simulink model "drone_plant"  (R2026a)
settings: Solver=ode4  StopTime=inf  FixedStep=P.Ts  RelTol=1e-8
PreLoadFcn:
  | model_params
values from neighbouring files (symbols this model uses):
  P = evalin('base','P')    [drone_panel.m]    (also in record_mission.m)
  x0 = zeros(12,1);  x0(3) = -3    [drone_panel.m]    (also in model_params.m = zeros(12,1); record_mission.m = zeros(12,1);  x0(3) = -P.field.alt)
undefined symbols (not defined in the file or in its folder): forces_islfcn, mixer_islfcn, obs_islfcn, plant_islfcn, pos_att_ctrl_islfcn, poserr_islfcn, sensors_islfcn, spray_islfcn, tilt_islfcn, traj_islfcn, wind_islfcn
settings Model: Creator=MALEK  LastModifiedBy=MALEK
settings SFSimCC: SimGPUStackLimitPerThread=51200
settings RTWCC: GPUStackLimitPerThread=51200

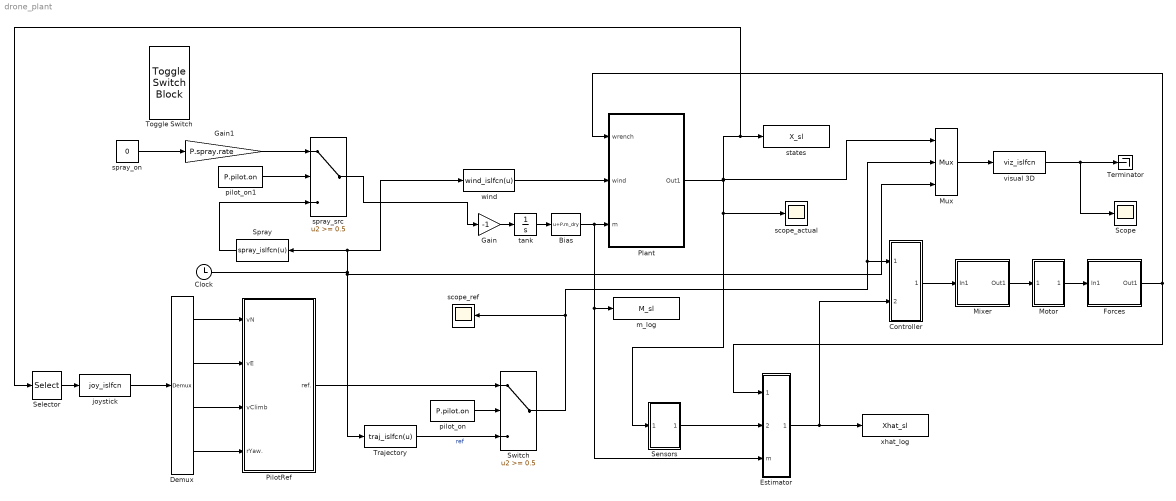
== system drone_plant ==
  Bias : Bias  Bias=P.m_dry  SaturateOnIntegerOverflow=off
  Clock : Clock
  Controller : Subsystem
  Demux : Demux
  Estimator : Subsystem
  Forces : Subsystem
  Gain : Gain  Gain=-1
  Gain1 : Gain  Gain=P.spray.rate
  Mixer : Subsystem
  "Motor  " : Subsystem
  Mux : Mux  Inputs=3
  PilotRef : Subsystem
  Plant : Subsystem
  Scope : Scope
      settings: ActiveDisplayYMinimum=-1  ActiveDisplayYMaximum=1  DataLoggingVariableName=ScopeData2
  Selector : Selector  InputPortWidth=12  IndexOptions=Index vector (dialog)  Indices=9  OutputSizes=1  RuntimeRangeChecks=off
  Sensors : Subsystem
  Spray : MATLABFcn  MATLABFcn=spray_islfcn(u)  OutputDimensions=1
  Switch : Switch  Threshold=0.5  SaturateOnIntegerOverflow=off  InputSameDT=off
  Terminator : Terminator
  Toggle Switch : ToggleSwitchBlock
  Trajectory : MATLABFcn  MATLABFcn=traj_islfcn(u)  OutputDimensions=10
  joystick : MATLABFcn  MATLABFcn=joy_islfcn  OutputDimensions=4
  m_log : ToWorkspace  VariableName=M_sl  SampleTime=-1
  pilot_on : Constant  Value=P.pilot.on
  pilot_on1 : Constant  Value=P.pilot.on
  scope_actual : Scope
      settings: ActiveDisplayYMinimum=-1  ActiveDisplayYMaximum=1
  scope_ref : Scope
      settings: ActiveDisplayYMinimum=-29.000000000000604  ActiveDisplayYMaximum=20.999999999998604
  spray_on : Constant  Value=0
  spray_src : Switch  Threshold=0.5  SaturateOnIntegerOverflow=off  InputSameDT=off
  states : ToWorkspace  VariableName=X_sl  SampleTime=-1
  tank : Integrator  InitialCondition=P.tank_full  LimitOutput=on  UpperSaturationLimit=P.tank_full  LowerSaturationLimit=0
  visual 3D : MATLABFcn  MATLABFcn=viz_islfcn  OutputDimensions=1
  wind : MATLABFcn  MATLABFcn=wind_islfcn(u)  OutputDimensions=3
  xhat_log : ToWorkspace  VariableName=Xhat_sl  SampleTime=-1
  wires:
  Estimator/1(Out1) -> xhat_log/1, Controller/2(In2)
  Sensors/1(Out1) -> Estimator/2(In2)
  Controller/1(Out1) -> Mixer/1(In1)
  Mixer/1(Out1) -> "Motor  "/1(In1)
  Forces/1(Out1) -> Estimator/1(In1), Plant/1(wrench)
  "Motor  "/1(Out1) -> Forces/1(In1)
  Clock/1 -> Trajectory/1, Mux/3, wind/1, Spray/1
  wind/1 -> Plant/2(wind)
  Spray/1 -> spray_src/3
  Gain/1 -> tank/1
  tank/1 -> Bias/1
  Bias/1 -> Estimator/3(m), m_log/1, Plant/3(m)
  PilotRef/1(ref.) -> Switch/1
  pilot_on/1 -> Switch/2
  Trajectory/1 -> Switch/3  "ref"
  Switch/1 -> Controller/1(In1), Mux/2, scope_ref/1
  spray_on/1 -> Gain1/1
  Gain1/1 -> spray_src/1
  spray_src/1 -> Gain/1
  pilot_on1/1 -> spray_src/2
  Mux/1 -> visual 3D/1
  visual 3D/1 -> Scope/1, Terminator/1
  Demux/4 -> PilotRef/4(rYaw.)
  Demux/3 -> PilotRef/3(vClimb)
  Demux/2 -> PilotRef/2(vE)
  Demux/1 -> PilotRef/1(vN)
  joystick/1 -> Demux/1
  Selector/1 -> joystick/1
  Plant/1(Out1) -> Mux/1, Selector/1, states/1, scope_actual/1, Sensors/1(In1)

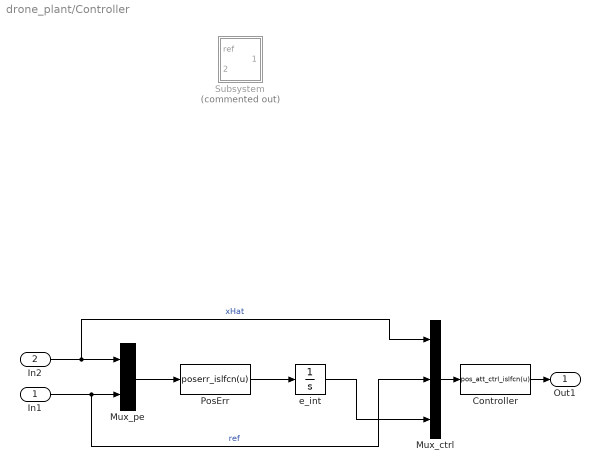
== system drone_plant/Controller ==
  In1 : Inport
  In2 : Inport  Port=2
  Controller : MATLABFcn  MATLABFcn=pos_att_ctrl_islfcn(u)  OutputDimensions=4
  Mux_ctrl : Mux  Inputs=3
  Mux_pe : Mux  Inputs=2
  PosErr : MATLABFcn  MATLABFcn=poserr_islfcn(u)  OutputDimensions=3
  Subsystem : Subsystem  Commented=on
  e_int : Integrator  LimitOutput=on  UpperSaturationLimit=P.int_limit  LowerSaturationLimit=-P.int_limit
  Out1 : Outport
  wires:
  In2/1 -> Mux_ctrl/1, Mux_pe/1  "xHat"
  In1/1 -> Mux_ctrl/2, Mux_pe/2  "ref"
  Mux_pe/1 -> PosErr/1
  PosErr/1 -> e_int/1
  e_int/1 -> Mux_ctrl/3
  Mux_ctrl/1 -> Controller/1
  Controller/1 -> Out1/1

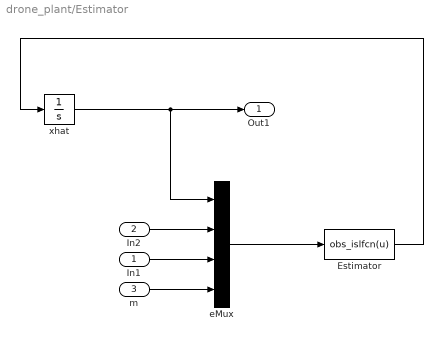
== system drone_plant/Estimator ==
  In1 : Inport
  In2 : Inport  Port=2
  m : Inport  Port=3
  Estimator : MATLABFcn  MATLABFcn=obs_islfcn(u)  OutputDimensions=12
  eMux : Mux
  xhat : Integrator  InitialCondition=x0
  Out1 : Outport
  wires:
  Estimator/1 -> xhat/1
  xhat/1 -> eMux/1, Out1/1
  In2/1 -> eMux/2
  eMux/1 -> Estimator/1
  In1/1 -> eMux/3
  m/1 -> eMux/4

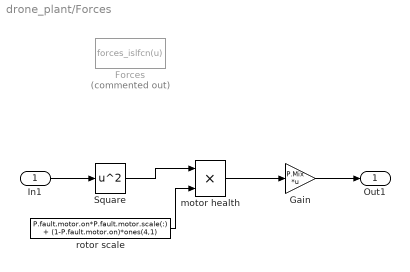
== system drone_plant/Forces ==
  In1 : Inport
  Forces : MATLABFcn  Commented=on  MATLABFcn=forces_islfcn(u)  OutputDimensions=4
  Gain : Gain  Gain=P.Mix  Multiplication=Matrix(K*u)
  Square : Math  Operator=square
  motor health : Product
  rotor scale : Constant  Value=P.fault.motor.on*P.fault.motor.scale(:) + (1-P.fault.motor.on)*ones(4,1)
  Out1 : Outport
  wires:
  In1/1 -> Square/1
  Gain/1 -> Out1/1
  Square/1 -> motor health/1
  rotor scale/1 -> motor health/2
  motor health/1 -> Gain/1

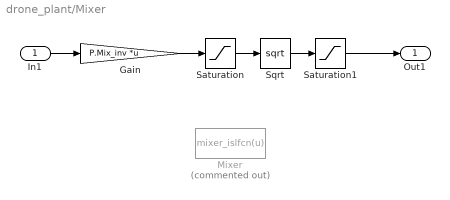
== system drone_plant/Mixer ==
  In1 : Inport
  Gain : Gain  Gain=P.Mix_inv  Multiplication=Matrix(K*u)
  Mixer : MATLABFcn  Commented=on  MATLABFcn=mixer_islfcn(u)  OutputDimensions=4
  Saturation : Saturate  UpperLimit=inf  LowerLimit=0
  Saturation1 : Saturate  UpperLimit=P.omega_max  LowerLimit=P.omega_min
  Sqrt : Sqrt
  Out1 : Outport
  wires:
  In1/1 -> Gain/1
  Gain/1 -> Saturation/1
  Saturation/1 -> Sqrt/1
  Sqrt/1 -> Saturation1/1
  Saturation1/1 -> Out1/1

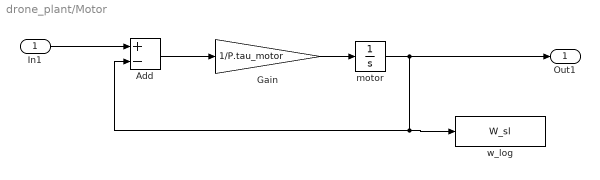
== system drone_plant/Motor   ==
  In1 : Inport
  Add : Sum  Inputs=+-
  Gain : Gain  Gain=1/P.tau_motor
  motor : Integrator  InitialCondition=P.omega_hover*ones(4,1)
  w_log : ToWorkspace  VariableName=W_sl  SampleTime=-1
  Out1 : Outport
  wires:
  In1/1 -> Add/1
  Gain/1 -> motor/1
  motor/1 -> w_log/1, Add/2, Out1/1
  Add/1 -> Gain/1

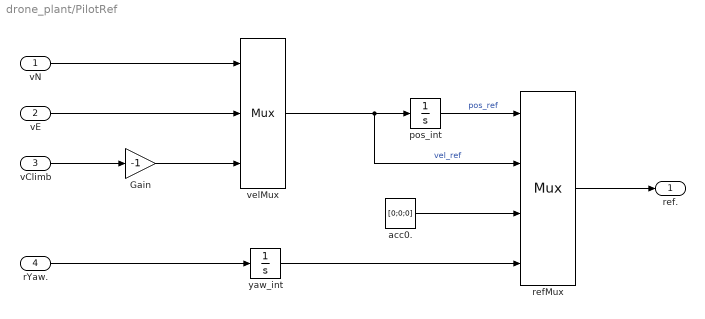
== system drone_plant/PilotRef ==
  vN : Inport
  vE : Inport  Port=2
  vClimb : Inport  Port=3
  rYaw. : Inport  Port=4
  Gain : Gain  Gain=-1
  acc0. : Constant  Value=[0;0;0]
  pos_int : Integrator  InitialCondition=x0(1:3)
  refMux : Mux
  velMux : Mux  Inputs=3
  yaw_int : Integrator  InitialCondition=x0(9)
  ref. : Outport
  wires:
  vClimb/1 -> Gain/1
  Gain/1 -> velMux/3
  vE/1 -> velMux/2
  vN/1 -> velMux/1
  velMux/1 -> refMux/2, pos_int/1  "vel_ref"
  rYaw./1 -> yaw_int/1
  pos_int/1 -> refMux/1  "pos_ref"
  acc0./1 -> refMux/3
  yaw_int/1 -> refMux/4
  refMux/1 -> ref./1

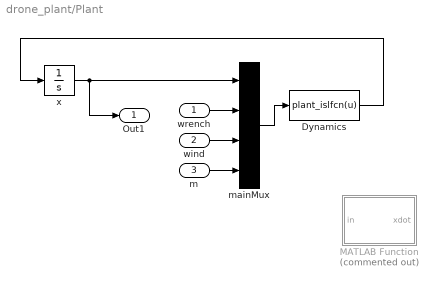
== system drone_plant/Plant ==
  wrench : Inport
  wind : Inport  Port=2
  m : Inport  Port=3
  Dynamics : MATLABFcn  MATLABFcn=plant_islfcn(u)  OutputDimensions=12
  MATLAB Function : MATLAB Function  Commented=on  TreatAsAtomicUnit=on
  mainMux : Mux
  x : Integrator  InitialCondition=x0
  Out1 : Outport
  wires:
  wrench/1 -> mainMux/2
  x/1 -> mainMux/1, Out1/1
  Dynamics/1 -> x/1
  mainMux/1 -> Dynamics/1
  wind/1 -> mainMux/3
  m/1 -> mainMux/4

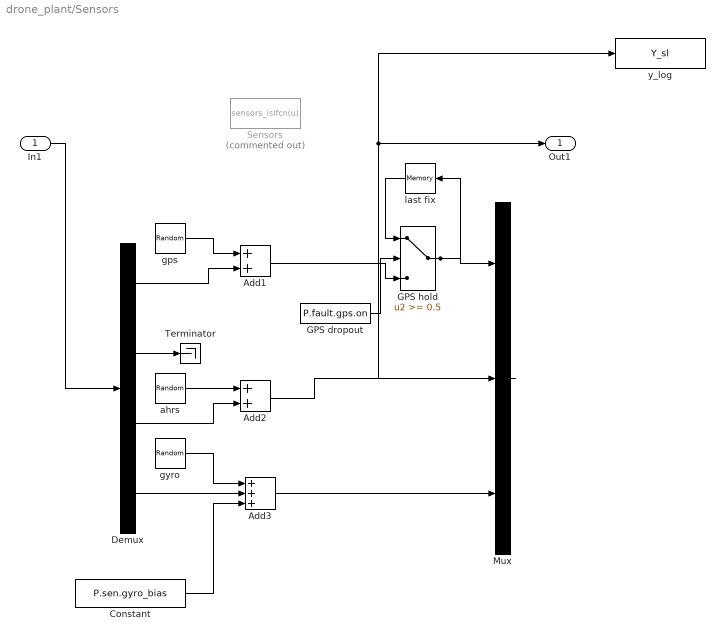
== system drone_plant/Sensors ==
  In1 : Inport
  Add1 : Sum
  Add2 : Sum
  Add3 : Sum  Inputs=+++
  Constant : Constant  Value=P.sen.gyro_bias
  Demux : Demux  Outputs=[3 3 3 3]
  GPS dropout : Constant  Value=P.fault.gps.on
  GPS hold : Switch  Threshold=0.5  SaturateOnIntegerOverflow=off  InputSameDT=off
  Mux : Mux  Inputs=3
  Sensors : MATLABFcn  Commented=on  MATLABFcn=sensors_islfcn(u)  OutputDimensions=9
  Terminator : Terminator
  ahrs : RandomNumber  Mean=[0;0;0]  Variance=P.sen.att_std^2  Seed=23456  SampleTime=P.Ts
  "gps " : RandomNumber  Mean=[0;0;0]  Variance=P.sen.gps_std^2  Seed=12345  SampleTime=P.Ts
  gyro : RandomNumber  Mean=[0;0;0]  Variance=P.sen.gyro_std^2  Seed=34567  SampleTime=P.Ts
  last fix : Memory
  y_log : ToWorkspace  VariableName=Y_sl  SampleTime=-1
  Out1 : Outport
  wires:
  In1/1 -> Demux/1
  Demux/2 -> Terminator/1
  "gps "/1 -> Add1/1
  Demux/1 -> Add1/2
  ahrs/1 -> Add2/1
  Demux/3 -> Add2/2
  gyro/1 -> Add3/1
  Demux/4 -> Add3/2
  Constant/1 -> Add3/3
  Add2/1 -> Mux/2
  Add3/1 -> Mux/3
  Mux/1 -> y_log/1, Out1/1
  Add1/1 -> GPS hold/3
  GPS dropout/1 -> GPS hold/2
  last fix/1 -> GPS hold/1
  GPS hold/1 -> last fix/1, Mux/1

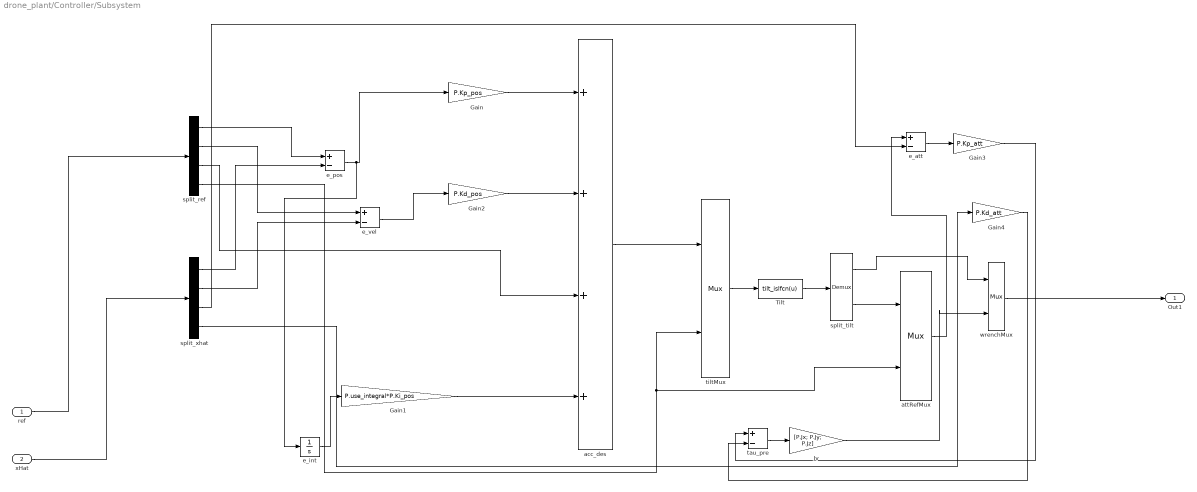
== system drone_plant/Controller/Subsystem ==
  ref : Inport
  xHat : Inport  Port=2
  Gain : Gain  Gain=P.Kp_pos
  Gain1 : Gain  Gain=P.use_integral*P.Ki_pos
  Gain2 : Gain  Gain=P.Kd_pos
  Gain3 : Gain  Gain=P.Kp_att
  Gain4 : Gain  Gain=P.Kd_att
  Jv : Gain  Gain=[P.Jx; P.Jy; P.Jz]
  Tilt : MATLABFcn  MATLABFcn=tilt_islfcn(u)  OutputDimensions=3
  acc_des : Sum  Inputs=++++
  attRefMux : Mux  Inputs=2
  e_att : Sum  Inputs=+-
  e_int : Integrator  LimitOutput=on  UpperSaturationLimit=P.int_limit  LowerSaturationLimit=-P.int_limit
  e_pos : Sum  Inputs=+-
  e_vel : Sum  Inputs=+-
  split_ref : Demux  Outputs=[3 3 3 1]
  split_tilt : Demux  Outputs=[1 2]
  split_xhat : Demux  Outputs=[3 3 3 3]
  tau_pre : Sum  Inputs=+-
  tiltMux : Mux  Inputs=2
  wrenchMux : Mux  Inputs=2
  Out1 : Outport
  wires:
  split_xhat/1 -> e_pos/2
  e_pos/1 -> e_int/1, Gain/1
  attRefMux/1 -> e_att/1
  split_xhat/3 -> e_att/2
  split_ref/3 -> acc_des/3
  Gain3/1 -> tau_pre/1
  e_att/1 -> Gain3/1
  e_vel/1 -> Gain2/1
  tau_pre/1 -> Jv/1
  split_xhat/2 -> e_vel/2
  split_tilt/2 -> attRefMux/1
  Gain/1 -> acc_des/1
  Tilt/1 -> split_tilt/1
  split_ref/4 -> attRefMux/2, tiltMux/2
  split_xhat/4 -> Gain4/1
  Gain1/1 -> acc_des/4
  split_ref/2 -> e_vel/1
  Jv/1 -> wrenchMux/2
  e_int/1 -> Gain1/1
  xHat/1 -> split_xhat/1
  split_ref/1 -> e_pos/1
  split_tilt/1 -> wrenchMux/1
  tiltMux/1 -> Tilt/1
  Gain2/1 -> acc_des/2
  Gain4/1 -> tau_pre/2
  acc_des/1 -> tiltMux/1
  ref/1 -> split_ref/1
  wrenchMux/1 -> Out1/1

== matlab function drone_plant/Plant/MATLAB Function ==
  data: in input; xdot output
function xdot = plant_islfcn(in)
%PLANT_ISLFCN  Simulink bridge to the verified quad_plant dynamics.
%   Driven by an "Interpreted MATLAB Function" block.
%   Input  in = [ x(1:12) ; u(13:16) ]   (state stacked on top of wrench)
%   Output xdot(12)
%   Runs in the BASE workspace, so the parameter struct P is fetched from there.
    P = evalin('base','P');
    x = in(1:12);
    u = in(13:16);
    if numel(in) >= 19, Fwind = in(17:19); else, Fwind = [0;0;0]; end
    if numel(in) >= 20, m_now = in(20);    else, m_now = P.m;     end
    xdot = quad_plant(0, x, u, P, Fwind, m_now);   % same function the oracle uses
end
